simulink model "sst_cllc_ttype_inv_discrete"  (R2026b)
settings: Solver=ode23tb  StopTime=simlength  FixedStep=tc  MaxStep=glb_time.tc
values from neighbouring files (symbols this model uses):
  param = sst_cllc_ttype_setup(param)    [init_model.m]
undefined symbols (not defined in the file or in its folder): afe_ctrl, glb_time, grid_emu, hwdata, omega_set, single_phase_inverter_ctrl, sst_num_of_modules
libraries: fl_lib x28, nesl_utility x16, discrete_time_low_pass_filter x4, lithium_ion_battery x2, cllc_dcx x2, dclink_for_three_levels x2, full_bridge_three_level_ttype_ideal_switch_based_model x2, full_bridge_three_level_ttype_mosfet_based_model x2, simulink x2, cstblocks_lti x2, single_phase_three_levels_PWM_modulator x2, dq_vector_pi x2
(part 2 of 3)

== system sst_cllc_ttype_inv_discrete/single_phase_inverter_modB/single phase afe ==
  gate_commands : Inport
  ideal_switch_based_three_level_inverter_ttype : full_bridge_three_level_ttype_ideal_switch_based_model/ideal_switch_based_three_level_inverter_ttype  Vth=ideal_switch.Vth  Ron=ideal_switch.Rds_on  Vdon_diode=ideal_switch.Vdon_diode  Rdon_diode=ideal_switch.Rdon_diode  Csnubber=ideal_switch.Csnubber  Rsnubber=ideal_switch.Rsnubber
  mosfet_based_three_level_inverter_ttype : full_bridge_three_level_ttype_mosfet_based_model/mosfet_based_three_level_inverter_ttype  Commented=on  Vth_m=mosfet.inv.Vth  Rds_on_m=mosfet.inv.Rds_on  Eon_m=mosfet.inv.Eon  Eoff_m=mosfet.inv.Eoff  Erec_m=mosfet.inv.Err  Ion_sw_loss_m=mosfet.inv.Ion_sw_losses  Voff_sw_loss_m=mosfet.inv.Voff_sw_losses  Vdon_diode_m=mosfet.inv.Vdon_diode  Rdon_diode_m=mosfet.inv.Rdon_diode  rth_mosfet_JH_m=mosfet.inv.Rth_mosfet_JH  rth_mosfet_HA_m=heatsink.Rth_mosfet_HA  Csnubber_m=mosfet.inv.Csnubber  Rsnubber_m=mosfet.inv.Rsnubber  JunctionTermalMass_m=mosfet.inv.JunctionTermalMass  mass_heatsink_m=heatsink.no_weight  specific_heat_m=heatsink.cp  Tambient_m=heatsink.Tambient  DThs_init_m=heatsink.DThs_init  tc_m=glb_time.tc
  references : Subsystem  Commented=on
  uac_out(+) : PMIOPort  Side=Left
  uac_out(-) : PMIOPort  Port=2  Side=Left
  udc(+) : PMIOPort  Port=3  Side=Right
  np : PMIOPort  Port=4  Side=Right
  udc(-) : PMIOPort  Port=5  Side=Right
  wires:
  mosfet_based_three_level_inverter_ttype/1 -> references/1(m)
  gate_commands/1 -> ideal_switch_based_three_level_inverter_ttype/1, mosfet_based_three_level_inverter_ttype/1
  connections:
  np/RConn1 -- mosfet_based_three_level_inverter_ttype/RConn2 -- ideal_switch_based_three_level_inverter_ttype/RConn2
  udc(-)/RConn1 -- mosfet_based_three_level_inverter_ttype/RConn3 -- ideal_switch_based_three_level_inverter_ttype/RConn3
  uac_out(+)/RConn1 -- mosfet_based_three_level_inverter_ttype/LConn1 -- ideal_switch_based_three_level_inverter_ttype/LConn1
  udc(+)/RConn1 -- mosfet_based_three_level_inverter_ttype/RConn1 -- ideal_switch_based_three_level_inverter_ttype/RConn1
  uac_out(-)/RConn1 -- mosfet_based_three_level_inverter_ttype/LConn2 -- ideal_switch_based_three_level_inverter_ttype/LConn2

== system sst_cllc_ttype_inv_discrete/single_phase_inverter_modB/single phase inverter control ==
  acquisition_and_scaling_current_with_white_noise : Subsystem
  acquisition_and_scaling_dc_voltage : Subsystem
  acquisition_and_scaling_grid_voltage_ac : Subsystem
  acquisition_and_scaling_voltage : Subsystem
  inverter_current_output_pu_reference : Subsystem
  pwm modulator : Subsystem
  single_phase_inverter_ctrl : Subsystem
  gate_cmds : Outport
  tag scope: afe_phase_grid_hat_modB=global
  wires:
  single_phase_inverter_ctrl/2(phase_grid_hat) -> [afe_phase_grid_hat_modB]
  acquisition_and_scaling_grid_voltage_ac/1(out) -> single_phase_inverter_ctrl/6(ugrid_pu)  "ug_abc"
  [ac_grid_voltage] -> acquisition_and_scaling_grid_voltage_ac/1(in)
  [time_afe_module_B] -> single_phase_inverter_ctrl/5(local_time)
  acquisition_and_scaling_dc_voltage/1(out) -> single_phase_inverter_ctrl/4(dclink_voltage_pu)  "dclink_voltage_pu"
  [dclink_voltage_modB] -> acquisition_and_scaling_dc_voltage/1(in)
  inverter_current_output_pu_reference/1(afe_current_output_pu_reference) -> single_phase_inverter_ctrl/3(afe_current output_pu_reference)  "afe_current_output_pu_reference"
  acquisition_and_scaling_voltage/1(out) -> single_phase_inverter_ctrl/1(afe_voltage_output_pu)  "afe_voltage_output_pu"
  acquisition_and_scaling_current_with_white_noise/1(out) -> single_phase_inverter_ctrl/2(afe_current_output_pu)  "afe_current_output_pu"
  single_phase_inverter_ctrl/1(u_ctrl_out) -> pwm modulator/1(vout)
  [afe_voltage_output_modB] -> acquisition_and_scaling_voltage/1(in)
  [TRGO_AFE_modB] -> single_phase_inverter_ctrl/Trigger
  pwm modulator/1(gate_cmds) -> gate_cmds/1
  [afe_is_modB] -> acquisition_and_scaling_current_with_white_noise/1(in)
  [udq_ctrl_out_modA] -> single_phase_inverter_ctrl/7(udq_ctrl_out)

== system sst_cllc_ttype_inv_discrete/single_phase_inverter_modA/dclink/references ==
  m : Inport
  Bus Selector : BusSelector  OutputSignals=udc,udc_p_gnd,udc_n_gnd,Cdc1_current
  Bus Selector1 : BusSelector  OutputSignals=idc1,idc2
  tag scope: CFi_dc_current_modA=global, dclink_n2gnd_voltage_modA=global, dclink_p2gnd_voltage_modA=global, dclink_voltage_modA=global, idc1_m_modA=global, idc2_m_modA=global
  wires:
  m/1 -> Bus Selector/1, Bus Selector1/1
  Bus Selector1/1 -> [idc1_m_modA]  "<idc1>"
  Bus Selector/1 -> [dclink_voltage_modA]  "<udc>"
  Bus Selector/4 -> [CFi_dc_current_modA]  "<Cdc1_current>"
  Bus Selector/3 -> [dclink_n2gnd_voltage_modA]  "<udc_n_gnd>"
  Bus Selector/2 -> [dclink_p2gnd_voltage_modA]  "<udc_p_gnd>"
  Bus Selector1/2 -> [idc2_m_modA]  "<idc2>"

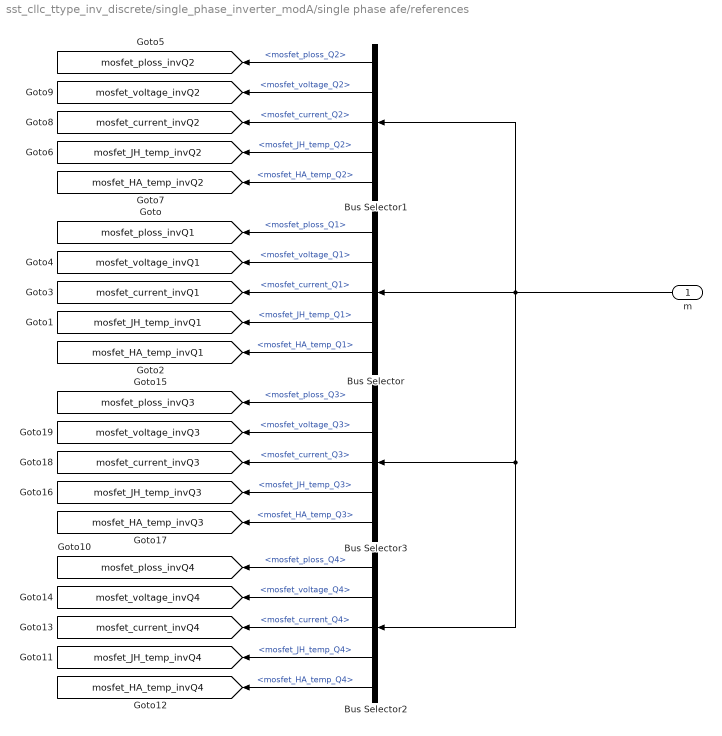
== system sst_cllc_ttype_inv_discrete/single_phase_inverter_modA/single phase afe/references ==
  m : Inport
  Bus Selector : BusSelector  OutputSignals=phaseleg_u.mosfet_ploss_Q1,phaseleg_u.mosfet_voltage_Q1,phaseleg_u.mosfet_current_Q1,phaseleg_u.mosfet_JH_temp_Q1,phaseleg_u.mosfet_HA_temp_Q1
  Bus Selector1 : BusSelector  OutputSignals=phaseleg_u.mosfet_ploss_Q2,phaseleg_u.mosfet_voltage_Q2,phaseleg_u.mosfet_current_Q2,phaseleg_u.mosfet_JH_temp_Q2,phaseleg_u.mosfet_HA_temp_Q2
  Bus Selector2 : BusSelector  OutputSignals=phaseleg_u.mosfet_ploss_Q4,phaseleg_u.mosfet_voltage_Q4,phaseleg_u.mosfet_current_Q4,phaseleg_u.mosfet_JH_temp_Q4,phaseleg_u.mosfet_HA_temp_Q4
  Bus Selector3 : BusSelector  OutputSignals=phaseleg_u.mosfet_ploss_Q3,phaseleg_u.mosfet_voltage_Q3,phaseleg_u.mosfet_current_Q3,phaseleg_u.mosfet_JH_temp_Q3,phaseleg_u.mosfet_HA_temp_Q3
  tag scope: mosfet_HA_temp_invQ1=global, mosfet_HA_temp_invQ2=global, mosfet_HA_temp_invQ3=global, mosfet_HA_temp_invQ4=global, mosfet_JH_temp_invQ1=global, mosfet_JH_temp_invQ2=global, mosfet_JH_temp_invQ3=global, mosfet_JH_temp_invQ4=global, mosfet_current_invQ1=global, mosfet_current_invQ2=global, mosfet_current_invQ3=global, mosfet_current_invQ4=global, mosfet_ploss_invQ1=global, mosfet_ploss_invQ2=global, mosfet_ploss_invQ3=global, mosfet_ploss_invQ4=global, mosfet_voltage_invQ1=global, mosfet_voltage_invQ2=global, mosfet_voltage_invQ3=global, mosfet_voltage_invQ4=global
  wires:
  Bus Selector/4 -> [mosfet_JH_temp_invQ1]  "<mosfet_JH_temp_Q1>"
  Bus Selector3/5 -> [mosfet_HA_temp_invQ3]  "<mosfet_HA_temp_Q3>"
  Bus Selector1/1 -> [mosfet_ploss_invQ2]  "<mosfet_ploss_Q2>"
  Bus Selector/5 -> [mosfet_HA_temp_invQ1]  "<mosfet_HA_temp_Q1>"
  Bus Selector/2 -> [mosfet_voltage_invQ1]  "<mosfet_voltage_Q1>"
  Bus Selector2/2 -> [mosfet_voltage_invQ4]  "<mosfet_voltage_Q4>"
  Bus Selector3/3 -> [mosfet_current_invQ3]  "<mosfet_current_Q3>"
  Bus Selector3/2 -> [mosfet_voltage_invQ3]  "<mosfet_voltage_Q3>"
  Bus Selector3/1 -> [mosfet_ploss_invQ3]  "<mosfet_ploss_Q3>"
  Bus Selector2/1 -> [mosfet_ploss_invQ4]  "<mosfet_ploss_Q4>"
  Bus Selector2/5 -> [mosfet_HA_temp_invQ4]  "<mosfet_HA_temp_Q4>"
  m/1 -> Bus Selector2/1, Bus Selector3/1, Bus Selector/1, Bus Selector1/1
  Bus Selector1/2 -> [mosfet_voltage_invQ2]  "<mosfet_voltage_Q2>"
  Bus Selector2/3 -> [mosfet_current_invQ4]  "<mosfet_current_Q4>"
  Bus Selector2/4 -> [mosfet_JH_temp_invQ4]  "<mosfet_JH_temp_Q4>"
  Bus Selector1/4 -> [mosfet_JH_temp_invQ2]  "<mosfet_JH_temp_Q2>"
  Bus Selector/1 -> [mosfet_ploss_invQ1]  "<mosfet_ploss_Q1>"
  Bus Selector1/3 -> [mosfet_current_invQ2]  "<mosfet_current_Q2>"
  Bus Selector3/4 -> [mosfet_JH_temp_invQ3]  "<mosfet_JH_temp_Q3>"
  Bus Selector/3 -> [mosfet_current_invQ1]  "<mosfet_current_Q1>"
  Bus Selector1/5 -> [mosfet_HA_temp_invQ2]  "<mosfet_HA_temp_Q2>"

== system sst_cllc_ttype_inv_discrete/single_phase_inverter_modA/single phase inverter control/acquisition_and_scaling_current ==
  in : Inport
  1/Ti5 : Gain  Gain=1/hwdata.single_phase_inverter.ibez  SaturateOnIntegerOverflow=on  OutDataTypeStr=Inherit: Same as input  ParamDataTypeStr=Inherit: Same as input
  Quantizer : Quantizer  QuantizationInterval=adc11_quantization
  out : Outport
  wires:
  Quantizer/1 -> out/1
  1/Ti5/1 -> Quantizer/1
  in/1 -> 1/Ti5/1

== system sst_cllc_ttype_inv_discrete/single_phase_inverter_modA/single phase inverter control/acquisition_and_scaling_current_with_white_noise ==
  in : Inport
  1/Ti5 : Gain  Gain=1/hwdata.single_phase_inverter.ibez  SaturateOnIntegerOverflow=on  OutDataTypeStr=Inherit: Same as input  ParamDataTypeStr=Inherit: Same as input
  Band-Limited White Noise : simulink/Sources/Band-Limited White Noise  Commented=on  Cov=1e-10  Ts=glb_time.tc  seed=[23341]
  Quantizer : Quantizer  QuantizationInterval=adc12_quantization
  Sum : Sum  Inputs=|++
  current_measure_with-without noise : Scope  NumInputPorts=2
      settings: ActiveDisplayYMinimum=-42.907449410116151  ActiveDisplayYMaximum=14.197534402303543  DataLoggingVariableName=ScopeData15
  out : Outport
  wires:
  1/Ti5/1 -> current_measure_with-without noise/1, Sum/1  "iload_without_noise"
  Sum/1 -> Quantizer/1
  Band-Limited White Noise/1 -> Sum/2
  Quantizer/1 -> out/1, current_measure_with-without noise/2  "iload_with_noise"
  in/1 -> 1/Ti5/1

== system sst_cllc_ttype_inv_discrete/single_phase_inverter_modA/single phase inverter control/acquisition_and_scaling_dc_voltage ==
  in : Inport
  1/Ti3 : Gain  Gain=1/hwdata.single_phase_inverter.udc_nom  SaturateOnIntegerOverflow=on  OutDataTypeStr=Inherit: Same as input  ParamDataTypeStr=Inherit: Same as input
  Quantizer : Quantizer  QuantizationInterval=adc12_quantization
  out : Outport
  wires:
  in/1 -> 1/Ti3/1
  1/Ti3/1 -> Quantizer/1
  Quantizer/1 -> out/1

== system sst_cllc_ttype_inv_discrete/single_phase_inverter_modA/single phase inverter control/acquisition_and_scaling_grid_voltage_ac ==
  in : Inport
  1/Ti1 : Gain  Gain=sst_num_of_modules  SaturateOnIntegerOverflow=on  OutDataTypeStr=Inherit: Same as input  ParamDataTypeStr=Inherit: Same as input
  1/Ti5 : Gain  Gain=1/grid_emu.u2bez  SaturateOnIntegerOverflow=on  OutDataTypeStr=Inherit: Same as input  ParamDataTypeStr=Inherit: Same as input
  Quantizer : Quantizer  QuantizationInterval=adc12_quantization
  out : Outport
  wires:
  Quantizer/1 -> out/1
  1/Ti5/1 -> Quantizer/1
  in/1 -> 1/Ti1/1
  1/Ti1/1 -> 1/Ti5/1

== system sst_cllc_ttype_inv_discrete/single_phase_inverter_modA/single phase inverter control/acquisition_and_scaling_voltage ==
  in : Inport
  1/Ti5 : Gain  Gain=1/hwdata.single_phase_inverter.ubez  SaturateOnIntegerOverflow=on  OutDataTypeStr=Inherit: Same as input  ParamDataTypeStr=Inherit: Same as input
  Quantizer : Quantizer  QuantizationInterval=adc12_quantization
  pwm filtering for measure : cstblocks_lti/LTI System  sys=sogi.flt.beta  IC=[]  PadeOrder=0
  out : Outport
  wires:
  in/1 -> 1/Ti5/1
  pwm filtering for measure/1 -> Quantizer/1
  1/Ti5/1 -> pwm filtering for measure/1
  Quantizer/1 -> out/1

== system sst_cllc_ttype_inv_discrete/single_phase_inverter_modA/single phase inverter control/inverter_current_output_pu_reference ==
  Rate Limiter : RateLimiter  RisingSlewLimit=param.spinv.i_ref_slew  FallingSlewLimit=-param.spinv.i_ref_slew  SampleTimeMode=inherited
  Step : Step  Time=param.spinv.t_ref  FinalValue=param.spinv.i_ref  SampleTime=0
  afe_current_output_pu_reference : Outport
  wires:
  Step/1 -> Rate Limiter/1
  Rate Limiter/1 -> afe_current_output_pu_reference/1

== system sst_cllc_ttype_inv_discrete/single_phase_inverter_modA/single phase inverter control/pwm modulator ==
  vout : Inport
  Constant : Constant  Value=0
  single_phase_three_levels_PWM_generator_with_global_TRGO : single_phase_three_levels_PWM_modulator/single_phase_three_levels_PWM_generator_with_global_TRGO  f=glb_time.fPWM_INV  m_up=1  m_low=-1  dead_time=glb_time.dead_time_AFE  pos_cmd_gate=15  neg_cmd_gate=-10  polarity=1  tc=glb_time.tc  double_sampling=glb_time.TRGO_AFE_double_update
  gate_cmds : Outport
  tag scope: TRGO_AFE_modA=global
  wires:
  vout/1 -> single_phase_three_levels_PWM_generator_with_global_TRGO/3
  Constant/1 -> single_phase_three_levels_PWM_generator_with_global_TRGO/2
  single_phase_three_levels_PWM_generator_with_global_TRGO/2 -> gate_cmds/1
  single_phase_three_levels_PWM_generator_with_global_TRGO/1 -> [TRGO_AFE_modA]
  [time_afe_module_A] -> single_phase_three_levels_PWM_generator_with_global_TRGO/1

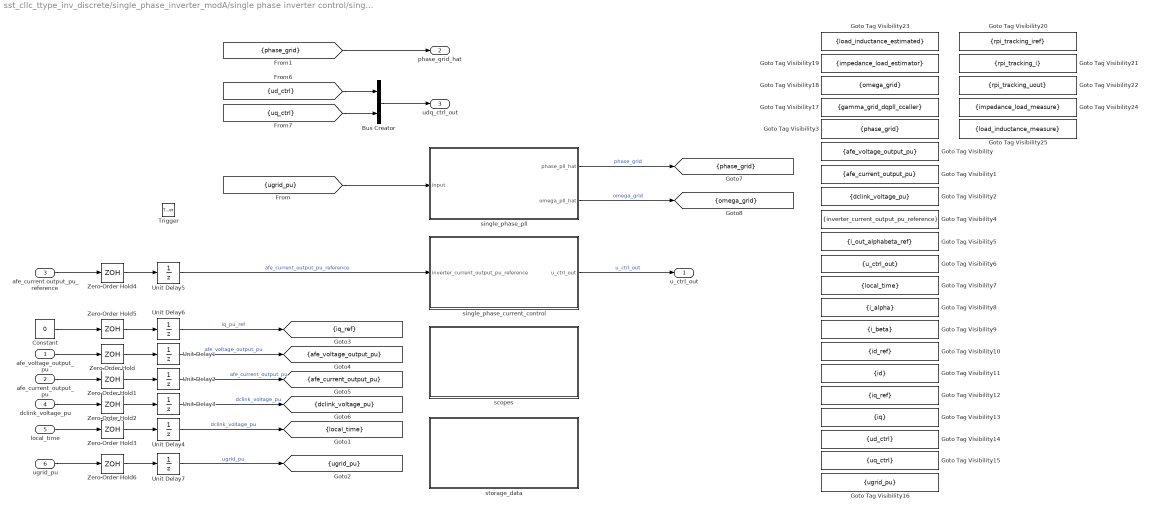
== system sst_cllc_ttype_inv_discrete/single_phase_inverter_modA/single phase inverter control/single_phase_inverter_ctrl ==
  afe_voltage_output_pu : Inport
  afe_current_output_pu : Inport  Port=2
  afe_current output_pu_reference : Inport  Port=3
  dclink_voltage_pu : Inport  Port=4
  local_time : Inport  Port=5
  ugrid_pu : Inport  Port=6
  Trigger : TriggerPort  VariantControl=(inherit)  PortDimensions=1
  Bus Creator : BusCreator  Inputs=2
  Constant : Constant  Value=0
  Goto Tag Visibility : GotoTagVisibility  GotoTag=afe_voltage_output_pu
  Goto Tag Visibility1 : GotoTagVisibility  GotoTag=afe_current_output_pu
  Goto Tag Visibility10 : GotoTagVisibility  GotoTag=id_ref
  Goto Tag Visibility11 : GotoTagVisibility  GotoTag=id
  Goto Tag Visibility12 : GotoTagVisibility  GotoTag=iq_ref
  Goto Tag Visibility13 : GotoTagVisibility  GotoTag=iq
  Goto Tag Visibility14 : GotoTagVisibility  GotoTag=ud_ctrl
  Goto Tag Visibility15 : GotoTagVisibility  GotoTag=uq_ctrl
  Goto Tag Visibility16 : GotoTagVisibility  GotoTag=ugrid_pu
  Goto Tag Visibility17 : GotoTagVisibility  GotoTag=gamma_grid_dqpll_ccaller
  Goto Tag Visibility18 : GotoTagVisibility  GotoTag=omega_grid
  Goto Tag Visibility19 : GotoTagVisibility  GotoTag=impedance_load_estimator
  Goto Tag Visibility2 : GotoTagVisibility  GotoTag=dclink_voltage_pu
  Goto Tag Visibility20 : GotoTagVisibility  GotoTag=rpi_tracking_iref
  Goto Tag Visibility21 : GotoTagVisibility  GotoTag=rpi_tracking_i
  Goto Tag Visibility22 : GotoTagVisibility  GotoTag=rpi_tracking_uout
  Goto Tag Visibility23 : GotoTagVisibility  GotoTag=load_inductance_estimated
  Goto Tag Visibility24 : GotoTagVisibility  GotoTag=impedance_load_measure
  Goto Tag Visibility25 : GotoTagVisibility  GotoTag=load_inductance_measure
  Goto Tag Visibility3 : GotoTagVisibility  GotoTag=phase_grid
  Goto Tag Visibility4 : GotoTagVisibility  GotoTag=inverter_current_output_pu_reference
  Goto Tag Visibility5 : GotoTagVisibility  GotoTag=i_out_alphabeta_ref
  Goto Tag Visibility6 : GotoTagVisibility  GotoTag=u_ctrl_out
  Goto Tag Visibility7 : GotoTagVisibility  GotoTag=local_time
  Goto Tag Visibility8 : GotoTagVisibility  GotoTag=i_alpha
  Goto Tag Visibility9 : GotoTagVisibility  GotoTag=i_beta
  Unit Delay{1..7} (7 alike) : UnitDelay  SampleTime=-1
  Zero-Order Hold{,1..6} (7 alike) : ZeroOrderHold  SampleTime=-1
  scopes : Subsystem
  single_phase_current_control : Subsystem
  single_phase_pll : Subsystem
  storage_data : Subsystem
  u_ctrl_out : Outport
  phase_grid_hat : Outport  Port=2
  udq_ctrl_out : Outport  Port=3
  tag scope: afe_current_output_pu=scoped, afe_voltage_output_pu=scoped, dclink_voltage_pu=scoped, iq_ref=scoped, local_time=scoped, omega_grid=scoped, phase_grid=scoped, ugrid_pu=scoped
  wires:
  afe_voltage_output_pu/1 -> Zero-Order Hold/1
  afe_current_output_pu/1 -> Zero-Order Hold1/1
  dclink_voltage_pu/1 -> Zero-Order Hold2/1
  Unit Delay1/1 -> [afe_voltage_output_pu]  "afe_voltage_output_pu"
  Unit Delay2/1 -> [afe_current_output_pu]  "afe_current_output_pu"
  Unit Delay3/1 -> [dclink_voltage_pu]  "dclink_voltage_pu"
  single_phase_pll/1(phase_pll_hat) -> [phase_grid]  "phase_grid"
  afe_current output_pu_reference/1 -> Zero-Order Hold4/1
  single_phase_current_control/1(u_ctrl_out) -> u_ctrl_out/1  "u_ctrl_out"
  Zero-Order Hold/1 -> Unit Delay1/1
  Zero-Order Hold1/1 -> Unit Delay2/1
  Zero-Order Hold2/1 -> Unit Delay3/1
  Zero-Order Hold3/1 -> Unit Delay4/1
  Unit Delay4/1 -> [local_time]  "dclink_voltage_pu"
  local_time/1 -> Zero-Order Hold3/1
  Zero-Order Hold4/1 -> Unit Delay5/1
  Unit Delay5/1 -> single_phase_current_control/1(inverter_current_output_pu_reference)  "afe_current_output_pu_reference"
  Constant/1 -> Zero-Order Hold5/1
  Zero-Order Hold5/1 -> Unit Delay6/1
  Unit Delay6/1 -> [iq_ref]  "iq_pu_ref"
  ugrid_pu/1 -> Zero-Order Hold6/1
  Zero-Order Hold6/1 -> Unit Delay7/1
  Unit Delay7/1 -> [ugrid_pu]  "ugrid_pu"
  single_phase_pll/2(omega_pll_hat) -> [omega_grid]  "omega_grid"
  [ugrid_pu] -> single_phase_pll/1(input)
  [phase_grid] -> phase_grid_hat/1
  Bus Creator/1 -> udq_ctrl_out/1
  [ud_ctrl] -> Bus Creator/1
  [uq_ctrl] -> Bus Creator/2

== system sst_cllc_ttype_inv_discrete/single_phase_inverter_modB/dclink/references ==
  m : Inport
  Bus Selector : BusSelector  OutputSignals=udc,udc_p_gnd,udc_n_gnd,Cdc1_current
  Bus Selector1 : BusSelector  OutputSignals=idc1,idc2
  tag scope: CFi_dc_current_modB=global, dclink_n2gnd_voltage_modB=global, dclink_p2gnd_voltage_modB=global, dclink_voltage_modB=global, idc1_m_modB=global, idc2_m_modB=global
  wires:
  Bus Selector1/2 -> [idc2_m_modB]  "<idc2>"
  Bus Selector/2 -> [dclink_p2gnd_voltage_modB]  "<udc_p_gnd>"
  Bus Selector/3 -> [dclink_n2gnd_voltage_modB]  "<udc_n_gnd>"
  Bus Selector/4 -> [CFi_dc_current_modB]  "<Cdc1_current>"
  Bus Selector/1 -> [dclink_voltage_modB]  "<udc>"
  Bus Selector1/1 -> [idc1_m_modB]  "<idc1>"
  m/1 -> Bus Selector1/1, Bus Selector/1

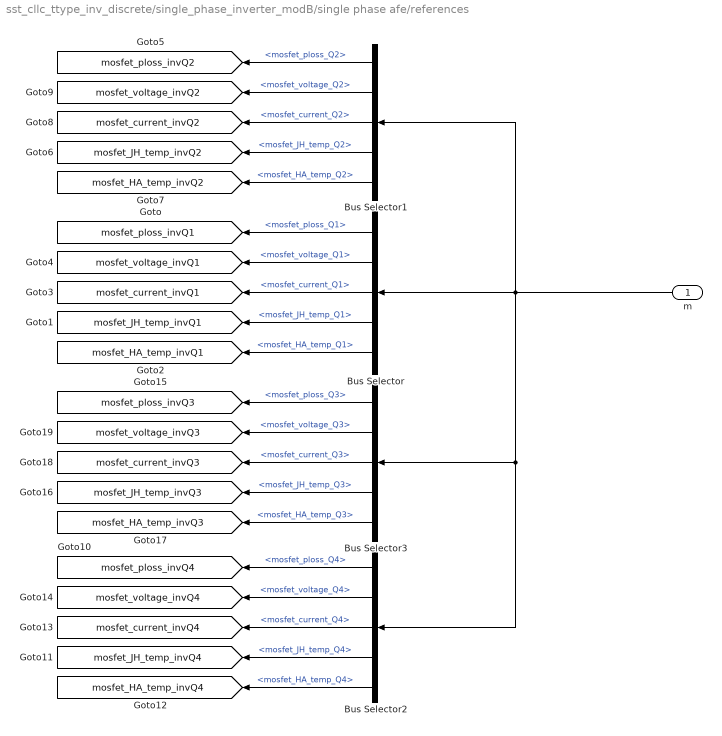
== system sst_cllc_ttype_inv_discrete/single_phase_inverter_modB/single phase afe/references ==
  m : Inport
  Bus Selector : BusSelector  OutputSignals=phaseleg_u.mosfet_ploss_Q1,phaseleg_u.mosfet_voltage_Q1,phaseleg_u.mosfet_current_Q1,phaseleg_u.mosfet_JH_temp_Q1,phaseleg_u.mosfet_HA_temp_Q1
  Bus Selector1 : BusSelector  OutputSignals=phaseleg_u.mosfet_ploss_Q2,phaseleg_u.mosfet_voltage_Q2,phaseleg_u.mosfet_current_Q2,phaseleg_u.mosfet_JH_temp_Q2,phaseleg_u.mosfet_HA_temp_Q2
  Bus Selector2 : BusSelector  OutputSignals=phaseleg_u.mosfet_ploss_Q4,phaseleg_u.mosfet_voltage_Q4,phaseleg_u.mosfet_current_Q4,phaseleg_u.mosfet_JH_temp_Q4,phaseleg_u.mosfet_HA_temp_Q4
  Bus Selector3 : BusSelector  OutputSignals=phaseleg_u.mosfet_ploss_Q3,phaseleg_u.mosfet_voltage_Q3,phaseleg_u.mosfet_current_Q3,phaseleg_u.mosfet_JH_temp_Q3,phaseleg_u.mosfet_HA_temp_Q3
  tag scope: mosfet_HA_temp_invQ1=global, mosfet_HA_temp_invQ2=global, mosfet_HA_temp_invQ3=global, mosfet_HA_temp_invQ4=global, mosfet_JH_temp_invQ1=global, mosfet_JH_temp_invQ2=global, mosfet_JH_temp_invQ3=global, mosfet_JH_temp_invQ4=global, mosfet_current_invQ1=global, mosfet_current_invQ2=global, mosfet_current_invQ3=global, mosfet_current_invQ4=global, mosfet_ploss_invQ1=global, mosfet_ploss_invQ2=global, mosfet_ploss_invQ3=global, mosfet_ploss_invQ4=global, mosfet_voltage_invQ1=global, mosfet_voltage_invQ2=global, mosfet_voltage_invQ3=global, mosfet_voltage_invQ4=global
  wires:
  Bus Selector1/5 -> [mosfet_HA_temp_invQ2]  "<mosfet_HA_temp_Q2>"
  Bus Selector/3 -> [mosfet_current_invQ1]  "<mosfet_current_Q1>"
  Bus Selector3/4 -> [mosfet_JH_temp_invQ3]  "<mosfet_JH_temp_Q3>"
  Bus Selector1/3 -> [mosfet_current_invQ2]  "<mosfet_current_Q2>"
  Bus Selector/1 -> [mosfet_ploss_invQ1]  "<mosfet_ploss_Q1>"
  Bus Selector1/4 -> [mosfet_JH_temp_invQ2]  "<mosfet_JH_temp_Q2>"
  Bus Selector2/4 -> [mosfet_JH_temp_invQ4]  "<mosfet_JH_temp_Q4>"
  Bus Selector2/3 -> [mosfet_current_invQ4]  "<mosfet_current_Q4>"
  Bus Selector1/2 -> [mosfet_voltage_invQ2]  "<mosfet_voltage_Q2>"
  m/1 -> Bus Selector1/1, Bus Selector/1, Bus Selector3/1, Bus Selector2/1
  Bus Selector2/5 -> [mosfet_HA_temp_invQ4]  "<mosfet_HA_temp_Q4>"
  Bus Selector2/1 -> [mosfet_ploss_invQ4]  "<mosfet_ploss_Q4>"
  Bus Selector3/1 -> [mosfet_ploss_invQ3]  "<mosfet_ploss_Q3>"
  Bus Selector3/2 -> [mosfet_voltage_invQ3]  "<mosfet_voltage_Q3>"
  Bus Selector3/3 -> [mosfet_current_invQ3]  "<mosfet_current_Q3>"
  Bus Selector2/2 -> [mosfet_voltage_invQ4]  "<mosfet_voltage_Q4>"
  Bus Selector/2 -> [mosfet_voltage_invQ1]  "<mosfet_voltage_Q1>"
  Bus Selector/5 -> [mosfet_HA_temp_invQ1]  "<mosfet_HA_temp_Q1>"
  Bus Selector1/1 -> [mosfet_ploss_invQ2]  "<mosfet_ploss_Q2>"
  Bus Selector3/5 -> [mosfet_HA_temp_invQ3]  "<mosfet_HA_temp_Q3>"
  Bus Selector/4 -> [mosfet_JH_temp_invQ1]  "<mosfet_JH_temp_Q1>"

== system sst_cllc_ttype_inv_discrete/single_phase_inverter_modB/single phase inverter control/acquisition_and_scaling_current_with_white_noise ==
  in : Inport
  1/Ti5 : Gain  Gain=1/hwdata.single_phase_inverter.ibez  SaturateOnIntegerOverflow=on  OutDataTypeStr=Inherit: Same as input  ParamDataTypeStr=Inherit: Same as input
  Band-Limited White Noise : simulink/Sources/Band-Limited White Noise  Commented=on  Cov=1e-10  Ts=glb_time.tc  seed=[23341]
  Quantizer : Quantizer  QuantizationInterval=adc12_quantization
  Sum : Sum  Inputs=|++
  current_measure_with-without noise : Scope  NumInputPorts=2
      settings: ActiveDisplayYMinimum=-42.907449410116151  ActiveDisplayYMaximum=14.197534402303543  DataLoggingVariableName=ScopeData15
  out : Outport
  wires:
  in/1 -> 1/Ti5/1
  Quantizer/1 -> current_measure_with-without noise/2, out/1  "iload_with_noise"
  Band-Limited White Noise/1 -> Sum/2
  Sum/1 -> Quantizer/1
  1/Ti5/1 -> Sum/1, current_measure_with-without noise/1  "iload_without_noise"

== system sst_cllc_ttype_inv_discrete/single_phase_inverter_modB/single phase inverter control/acquisition_and_scaling_dc_voltage ==
  in : Inport
  1/Ti3 : Gain  Gain=1/hwdata.single_phase_inverter.udc_nom  SaturateOnIntegerOverflow=on  OutDataTypeStr=Inherit: Same as input  ParamDataTypeStr=Inherit: Same as input
  Quantizer : Quantizer  QuantizationInterval=adc12_quantization
  out : Outport
  wires:
  Quantizer/1 -> out/1
  1/Ti3/1 -> Quantizer/1
  in/1 -> 1/Ti3/1

== system sst_cllc_ttype_inv_discrete/single_phase_inverter_modB/single phase inverter control/acquisition_and_scaling_grid_voltage_ac ==
  in : Inport
  1/Ti1 : Gain  Gain=sst_num_of_modules  SaturateOnIntegerOverflow=on  OutDataTypeStr=Inherit: Same as input  ParamDataTypeStr=Inherit: Same as input
  1/Ti5 : Gain  Gain=1/grid_emu.u2bez  SaturateOnIntegerOverflow=on  OutDataTypeStr=Inherit: Same as input  ParamDataTypeStr=Inherit: Same as input
  Quantizer : Quantizer  QuantizationInterval=adc12_quantization
  out : Outport
  wires:
  in/1 -> 1/Ti1/1
  1/Ti5/1 -> Quantizer/1
  Quantizer/1 -> out/1
  1/Ti1/1 -> 1/Ti5/1

== system sst_cllc_ttype_inv_discrete/single_phase_inverter_modB/single phase inverter control/acquisition_and_scaling_voltage ==
  in : Inport
  1/Ti5 : Gain  Gain=1/hwdata.single_phase_inverter.ubez  SaturateOnIntegerOverflow=on  OutDataTypeStr=Inherit: Same as input  ParamDataTypeStr=Inherit: Same as input
  Quantizer : Quantizer  QuantizationInterval=adc12_quantization
  pwm filtering for measure : cstblocks_lti/LTI System  sys=sogi.flt.beta  IC=[]  PadeOrder=0
  out : Outport
  wires:
  Quantizer/1 -> out/1
  1/Ti5/1 -> pwm filtering for measure/1
  pwm filtering for measure/1 -> Quantizer/1
  in/1 -> 1/Ti5/1

== system sst_cllc_ttype_inv_discrete/single_phase_inverter_modB/single phase inverter control/inverter_current_output_pu_reference ==
  Constant : Constant  Value=param.spinv.i_ref
  afe_current_output_pu_reference : Outport
  wires:
  Constant/1 -> afe_current_output_pu_reference/1

== system sst_cllc_ttype_inv_discrete/single_phase_inverter_modB/single phase inverter control/pwm modulator ==
  vout : Inport
  Constant : Constant  Value=0
  single_phase_three_levels_PWM_generator_with_global_TRGO : single_phase_three_levels_PWM_modulator/single_phase_three_levels_PWM_generator_with_global_TRGO  f=glb_time.fPWM_INV  m_up=1  m_low=-1  dead_time=glb_time.dead_time_AFE  pos_cmd_gate=15  neg_cmd_gate=-10  polarity=1  tc=glb_time.tc  double_sampling=glb_time.TRGO_AFE_double_update
  gate_cmds : Outport
  tag scope: TRGO_AFE_modB=global
  wires:
  [time_afe_module_B] -> single_phase_three_levels_PWM_generator_with_global_TRGO/1
  single_phase_three_levels_PWM_generator_with_global_TRGO/1 -> [TRGO_AFE_modB]
  single_phase_three_levels_PWM_generator_with_global_TRGO/2 -> gate_cmds/1
  Constant/1 -> single_phase_three_levels_PWM_generator_with_global_TRGO/2
  vout/1 -> single_phase_three_levels_PWM_generator_with_global_TRGO/3

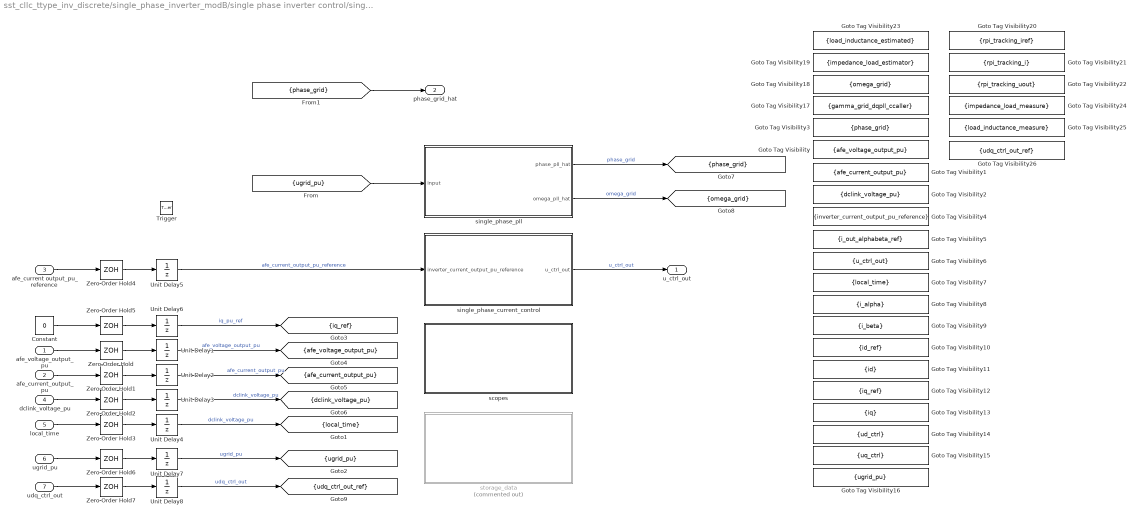
== system sst_cllc_ttype_inv_discrete/single_phase_inverter_modB/single phase inverter control/single_phase_inverter_ctrl ==
  afe_voltage_output_pu : Inport
  afe_current_output_pu : Inport  Port=2
  afe_current output_pu_reference : Inport  Port=3
  dclink_voltage_pu : Inport  Port=4
  local_time : Inport  Port=5
  ugrid_pu : Inport  Port=6
  udq_ctrl_out : Inport  Port=7
  Trigger : TriggerPort  VariantControl=(inherit)  PortDimensions=1
  Constant : Constant  Value=0
  Goto Tag Visibility : GotoTagVisibility  GotoTag=afe_voltage_output_pu
  Goto Tag Visibility1 : GotoTagVisibility  GotoTag=afe_current_output_pu
  Goto Tag Visibility10 : GotoTagVisibility  GotoTag=id_ref
  Goto Tag Visibility11 : GotoTagVisibility  GotoTag=id
  Goto Tag Visibility12 : GotoTagVisibility  GotoTag=iq_ref
  Goto Tag Visibility13 : GotoTagVisibility  GotoTag=iq
  Goto Tag Visibility14 : GotoTagVisibility  GotoTag=ud_ctrl
  Goto Tag Visibility15 : GotoTagVisibility  GotoTag=uq_ctrl
  Goto Tag Visibility16 : GotoTagVisibility  GotoTag=ugrid_pu
  Goto Tag Visibility17 : GotoTagVisibility  GotoTag=gamma_grid_dqpll_ccaller
  Goto Tag Visibility18 : GotoTagVisibility  GotoTag=omega_grid
  Goto Tag Visibility19 : GotoTagVisibility  GotoTag=impedance_load_estimator
  Goto Tag Visibility2 : GotoTagVisibility  GotoTag=dclink_voltage_pu
  Goto Tag Visibility20 : GotoTagVisibility  GotoTag=rpi_tracking_iref
  Goto Tag Visibility21 : GotoTagVisibility  GotoTag=rpi_tracking_i
  Goto Tag Visibility22 : GotoTagVisibility  GotoTag=rpi_tracking_uout
  Goto Tag Visibility23 : GotoTagVisibility  GotoTag=load_inductance_estimated
  Goto Tag Visibility24 : GotoTagVisibility  GotoTag=impedance_load_measure
  Goto Tag Visibility25 : GotoTagVisibility  GotoTag=load_inductance_measure
  Goto Tag Visibility26 : GotoTagVisibility  GotoTag=udq_ctrl_out_ref
  Goto Tag Visibility3 : GotoTagVisibility  GotoTag=phase_grid
  Goto Tag Visibility4 : GotoTagVisibility  GotoTag=inverter_current_output_pu_reference
  Goto Tag Visibility5 : GotoTagVisibility  GotoTag=i_out_alphabeta_ref
  Goto Tag Visibility6 : GotoTagVisibility  GotoTag=u_ctrl_out
  Goto Tag Visibility7 : GotoTagVisibility  GotoTag=local_time
  Goto Tag Visibility8 : GotoTagVisibility  GotoTag=i_alpha
  Goto Tag Visibility9 : GotoTagVisibility  GotoTag=i_beta
  Unit Delay{1..8} (8 alike) : UnitDelay  SampleTime=-1
  Zero-Order Hold{,1..7} (8 alike) : ZeroOrderHold  SampleTime=-1
  scopes : Subsystem
  single_phase_current_control : Subsystem
  single_phase_pll : Subsystem
  storage_data : Subsystem  Commented=on
  u_ctrl_out : Outport
  phase_grid_hat : Outport  Port=2
  tag scope: afe_current_output_pu=scoped, afe_voltage_output_pu=scoped, dclink_voltage_pu=scoped, iq_ref=scoped, local_time=scoped, omega_grid=scoped, phase_grid=scoped, udq_ctrl_out_ref=scoped, ugrid_pu=scoped
  wires:
  [phase_grid] -> phase_grid_hat/1
  [ugrid_pu] -> single_phase_pll/1(input)
  single_phase_pll/2(omega_pll_hat) -> [omega_grid]  "omega_grid"
  Unit Delay7/1 -> [ugrid_pu]  "ugrid_pu"
  Zero-Order Hold6/1 -> Unit Delay7/1
  ugrid_pu/1 -> Zero-Order Hold6/1
  Unit Delay6/1 -> [iq_ref]  "iq_pu_ref"
  Zero-Order Hold5/1 -> Unit Delay6/1
  Constant/1 -> Zero-Order Hold5/1
  Unit Delay5/1 -> single_phase_current_control/1(inverter_current_output_pu_reference)  "afe_current_output_pu_reference"
  Zero-Order Hold4/1 -> Unit Delay5/1
  local_time/1 -> Zero-Order Hold3/1
  Unit Delay4/1 -> [local_time]  "dclink_voltage_pu"
  Zero-Order Hold3/1 -> Unit Delay4/1
  Zero-Order Hold2/1 -> Unit Delay3/1
  Zero-Order Hold1/1 -> Unit Delay2/1
  Zero-Order Hold/1 -> Unit Delay1/1
  single_phase_current_control/1(u_ctrl_out) -> u_ctrl_out/1  "u_ctrl_out"
  afe_current output_pu_reference/1 -> Zero-Order Hold4/1
  single_phase_pll/1(phase_pll_hat) -> [phase_grid]  "phase_grid"
  Unit Delay3/1 -> [dclink_voltage_pu]  "dclink_voltage_pu"
  Unit Delay2/1 -> [afe_current_output_pu]  "afe_current_output_pu"
  Unit Delay1/1 -> [afe_voltage_output_pu]  "afe_voltage_output_pu"
  dclink_voltage_pu/1 -> Zero-Order Hold2/1
  afe_current_output_pu/1 -> Zero-Order Hold1/1
  afe_voltage_output_pu/1 -> Zero-Order Hold/1
  udq_ctrl_out/1 -> Zero-Order Hold7/1
  Zero-Order Hold7/1 -> Unit Delay8/1
  Unit Delay8/1 -> [udq_ctrl_out_ref]  "udq_ctrl_out"

== system sst_cllc_ttype_inv_discrete/single_phase_inverter_modA/single phase inverter control/single_phase_inverter_ctrl/scopes ==
  Bus Creator1 : BusCreator  Inputs=3
  Bus Creator2 : BusCreator  Inputs=2
  Bus Creator3 : BusCreator  Inputs=2
  Bus Creator4 : BusCreator  Inputs=2
  single phase inverter tracking current scope 1 : Scope  NumInputPorts=2
      settings: ActiveDisplayYMinimum=-0.98089599609375  ActiveDisplayYMaximum=0.98138427734375  DataLoggingVariableName=ScopeData12
  single phase inverter tracking current scope 2 : Scope  NumInputPorts=2
      settings: ActiveDisplayYMinimum=-1.2603759765625  ActiveDisplayYMaximum=1.2652587890625  DataLoggingVariableName=ScopeData2
  wires:
  Bus Creator1/1 -> single phase inverter tracking current scope 1/2  "is_tracking"
  [i_out_alphabeta_ref] -> Bus Creator1/2  "i_out_inverter_pu_ref"
  [afe_current_output_pu] -> Bus Creator1/3  "inverter_current_output_pu"
  [afe_voltage_output_pu] -> Bus Creator2/1  "inverter_voltage_output_pu"
  Bus Creator2/1 -> single phase inverter tracking current scope 1/1  "load"
  [inverter_current_output_pu_reference] -> Bus Creator1/1  "inverter_current_output_pu_reference"
  [afe_current_output_pu] -> Bus Creator2/2  "inverter_current_output_pu"
  [u_ctrl_out] -> Bus Creator3/1  "u_ctrl_out"
  [afe_voltage_output_pu] -> Bus Creator3/2  "inverter_voltage_output_pu"
  Bus Creator3/1 -> single phase inverter tracking current scope 2/2  "u_load"
  [afe_current_output_pu] -> Bus Creator4/2  "inverter_current_output_pu"
  [i_out_alphabeta_ref] -> Bus Creator4/1  "i_out_alphabeta_ref"
  Bus Creator4/1 -> single phase inverter tracking current scope 2/1  "i_load"

== system sst_cllc_ttype_inv_discrete/single_phase_inverter_modA/single phase inverter control/single_phase_inverter_ctrl/single_phase_current_control ==
  inverter_current_output_pu_reference : Inport
  current_reference_generation : Subsystem
  dqpi_current_controller : Subsystem
  u_ctrl_out : Outport
  tag scope: i_out_alphabeta_ref=scoped, inverter_current_output_pu_reference=scoped, u_ctrl_out=scoped
  wires:
  current_reference_generation/1(is_ref) -> [i_out_alphabeta_ref]  "i_out_inverter_pu_ref"
  dqpi_current_controller/1(u_out) -> u_ctrl_out/1, [u_ctrl_out]  "u_ctrl_out"
  [phase_grid] -> current_reference_generation/2(phase)
  inverter_current_output_pu_reference/1 -> current_reference_generation/1(mag_ref), [inverter_current_output_pu_reference]
  current_reference_generation/2(id_ref) -> dqpi_current_controller/1(id_ref)

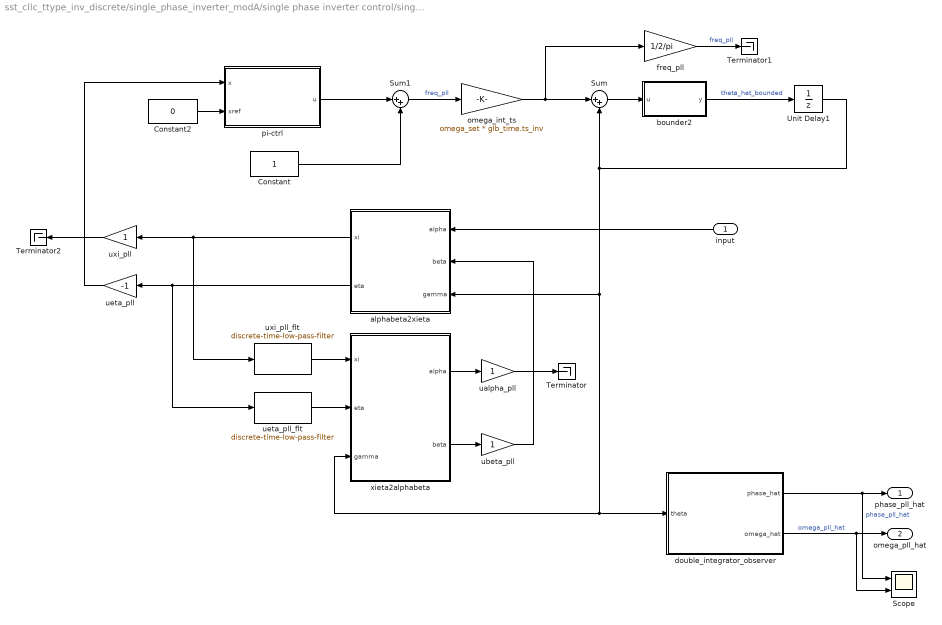
== system sst_cllc_ttype_inv_discrete/single_phase_inverter_modA/single phase inverter control/single_phase_inverter_ctrl/single_phase_pll ==
  input : Inport
  Constant : Constant
  Constant2 : Constant  Value=0
  Scope : Scope  NumInputPorts=2
      settings: ActiveDisplayYMinimum=-3.8846913322397336  ActiveDisplayYMaximum=3.9201093626393169
  Sum : Sum  Inputs=|++
  Sum1 : Sum  Inputs=|++
  Terminator : Terminator
  Terminator1 : Terminator
  Terminator2 : Terminator
  Unit Delay1 : UnitDelay  SampleTime=-1
  alphabeta2xieta : MATLAB Function  TreatAsAtomicUnit=on
  bounder2 : MATLAB Function  TreatAsAtomicUnit=on
  double_integrator_observer : Subsystem
  freq_pll : Gain  Gain=1/2/pi
  omega_int_ts : Gain  Gain=omega_set * glb_time.ts_inv
  pi-ctrl : Subsystem  mask{kp=1, ki=0, ts=glb_time.ts_inv, sat_pos=2, sat_neg=-2}
  ualpha_pll : Gain
  ubeta_pll : Gain
  ueta_pll : Gain  Gain=-1
  ueta_pll_flt : discrete_time_low_pass_filter/discrete-time-low-pass-filter  tau=2/omega_set  ts=glb_time.ts_inv
  uxi_pll : Gain
  uxi_pll_flt : discrete_time_low_pass_filter/discrete-time-low-pass-filter  tau=2/omega_set  ts=glb_time.ts_inv
  xieta2alphabeta : MATLAB Function  TreatAsAtomicUnit=on
  phase_pll_hat : Outport
  omega_pll_hat : Outport  Port=2
  wires:
  Sum/1 -> bounder2/1(u)
  alphabeta2xieta/1(xi) -> uxi_pll/1, uxi_pll_flt/1
  xieta2alphabeta/2(beta) -> ubeta_pll/1
  alphabeta2xieta/2(eta) -> ueta_pll/1, ueta_pll_flt/1
  omega_int_ts/1 -> freq_pll/1, Sum/1
  double_integrator_observer/1(phase_hat) -> Scope/1, phase_pll_hat/1  "phase_pll_hat"
  input/1 -> alphabeta2xieta/1(alpha)
  freq_pll/1 -> Terminator1/1  "freq_pll"
  ueta_pll_flt/1 -> xieta2alphabeta/2(eta)
  uxi_pll_flt/1 -> xieta2alphabeta/1(xi)
  ueta_pll/1 -> pi-ctrl/1(x)
  Sum1/1 -> omega_int_ts/1  "freq_pll"
  Constant2/1 -> pi-ctrl/2(xref)
  uxi_pll/1 -> Terminator2/1
  ubeta_pll/1 -> alphabeta2xieta/2(beta)
  xieta2alphabeta/1(alpha) -> ualpha_pll/1
  pi-ctrl/1(u) -> Sum1/1
  Constant/1 -> Sum1/2
  Unit Delay1/1 -> Sum/2, alphabeta2xieta/3(gamma), xieta2alphabeta/3(gamma), double_integrator_observer/1(theta)
  bounder2/1(y) -> Unit Delay1/1  "theta_hat_bounded"
  double_integrator_observer/2(omega_hat) -> Scope/2, omega_pll_hat/1  "omega_pll_hat"
  ualpha_pll/1 -> Terminator/1

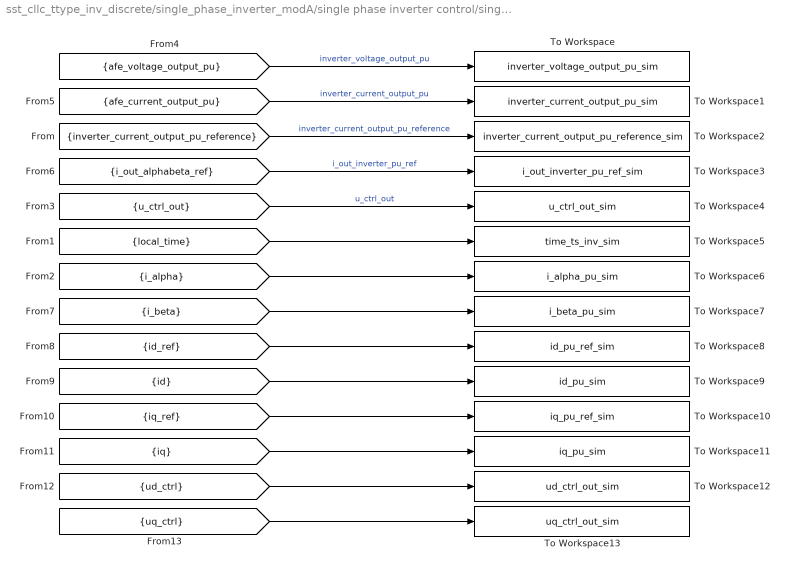
== system sst_cllc_ttype_inv_discrete/single_phase_inverter_modA/single phase inverter control/single_phase_inverter_ctrl/storage_data ==
  To Workspace : ToWorkspace  VariableName=inverter_voltage_output_pu_sim  SampleTime=-1
      settings: MaxDataPoints=glb_time.Ns_inv  Save2DSignal=2-D array (concatenate along first dimension)
  To Workspace1 : ToWorkspace  VariableName=inverter_current_output_pu_sim  SampleTime=-1
      settings: MaxDataPoints=glb_time.Ns_inv  Save2DSignal=2-D array (concatenate along first dimension)
  To Workspace10 : ToWorkspace  VariableName=iq_pu_ref_sim  SampleTime=-1
      settings: MaxDataPoints=glb_time.Ns_inv  Save2DSignal=2-D array (concatenate along first dimension)
  To Workspace11 : ToWorkspace  VariableName=iq_pu_sim  SampleTime=-1
      settings: MaxDataPoints=glb_time.Ns_inv  Save2DSignal=2-D array (concatenate along first dimension)
  To Workspace12 : ToWorkspace  VariableName=ud_ctrl_out_sim  SampleTime=-1
      settings: MaxDataPoints=glb_time.Ns_inv  Save2DSignal=2-D array (concatenate along first dimension)
  To Workspace13 : ToWorkspace  VariableName=uq_ctrl_out_sim  SampleTime=-1
      settings: MaxDataPoints=glb_time.Ns_inv  Save2DSignal=2-D array (concatenate along first dimension)
  To Workspace2 : ToWorkspace  VariableName=inverter_current_output_pu_reference_sim  SampleTime=-1
      settings: MaxDataPoints=glb_time.Ns_inv  Save2DSignal=2-D array (concatenate along first dimension)
  To Workspace3 : ToWorkspace  VariableName=i_out_inverter_pu_ref_sim  SampleTime=-1
      settings: MaxDataPoints=glb_time.Ns_inv  Save2DSignal=2-D array (concatenate along first dimension)
  To Workspace4 : ToWorkspace  VariableName=u_ctrl_out_sim  SampleTime=-1
      settings: MaxDataPoints=glb_time.Ns_inv  Save2DSignal=2-D array (concatenate along first dimension)
  To Workspace5 : ToWorkspace  VariableName=time_ts_inv_sim  SampleTime=-1
      settings: MaxDataPoints=glb_time.Ns_inv  Save2DSignal=2-D array (concatenate along first dimension)
  To Workspace6 : ToWorkspace  VariableName=i_alpha_pu_sim  SampleTime=-1
      settings: MaxDataPoints=glb_time.Ns_inv  Save2DSignal=2-D array (concatenate along first dimension)
  To Workspace7 : ToWorkspace  VariableName=i_beta_pu_sim  SampleTime=-1
      settings: MaxDataPoints=glb_time.Ns_inv  Save2DSignal=2-D array (concatenate along first dimension)
  To Workspace8 : ToWorkspace  VariableName=id_pu_ref_sim  SampleTime=-1
      settings: MaxDataPoints=glb_time.Ns_inv  Save2DSignal=2-D array (concatenate along first dimension)
  To Workspace9 : ToWorkspace  VariableName=id_pu_sim  SampleTime=-1
      settings: MaxDataPoints=glb_time.Ns_inv  Save2DSignal=2-D array (concatenate along first dimension)
  wires:
  [afe_voltage_output_pu] -> To Workspace/1  "inverter_voltage_output_pu"
  [afe_current_output_pu] -> To Workspace1/1  "inverter_current_output_pu"
  [inverter_current_output_pu_reference] -> To Workspace2/1  "inverter_current_output_pu_reference"
  [i_out_alphabeta_ref] -> To Workspace3/1  "i_out_inverter_pu_ref"
  [u_ctrl_out] -> To Workspace4/1  "u_ctrl_out"
  [local_time] -> To Workspace5/1
  [i_alpha] -> To Workspace6/1
  [i_beta] -> To Workspace7/1
  [id_ref] -> To Workspace8/1
  [id] -> To Workspace9/1
  [iq_ref] -> To Workspace10/1
  [iq] -> To Workspace11/1
  [ud_ctrl] -> To Workspace12/1
  [uq_ctrl] -> To Workspace13/1

== system sst_cllc_ttype_inv_discrete/single_phase_inverter_modB/single phase inverter control/single_phase_inverter_ctrl/scopes ==
  Bus Creator1 : BusCreator  Inputs=3
  Bus Creator2 : BusCreator  Inputs=2
  Bus Creator3 : BusCreator  Inputs=2
  Bus Creator4 : BusCreator  Inputs=2
  single phase inverter tracking current scope 1 : Scope  NumInputPorts=2
      settings: ActiveDisplayYMinimum=-1.23468017578125  ActiveDisplayYMaximum=1.23419189453125  DataLoggingVariableName=ScopeData12
  single phase inverter tracking current scope 2 : Scope  NumInputPorts=2
      settings: ActiveDisplayYMinimum=-1.2603759765625  ActiveDisplayYMaximum=1.2652587890625  DataLoggingVariableName=ScopeData2
  wires:
  Bus Creator4/1 -> single phase inverter tracking current scope 2/1  "i_load"
  [i_out_alphabeta_ref] -> Bus Creator4/1  "i_out_alphabeta_ref"
  [afe_current_output_pu] -> Bus Creator4/2  "inverter_current_output_pu"
  Bus Creator3/1 -> single phase inverter tracking current scope 2/2  "u_load"
  [afe_voltage_output_pu] -> Bus Creator3/2  "inverter_voltage_output_pu"
  [u_ctrl_out] -> Bus Creator3/1  "u_ctrl_out"
  [afe_current_output_pu] -> Bus Creator2/2  "inverter_current_output_pu"
  [inverter_current_output_pu_reference] -> Bus Creator1/1  "inverter_current_output_pu_reference"
  Bus Creator2/1 -> single phase inverter tracking current scope 1/1  "load"
  [afe_voltage_output_pu] -> Bus Creator2/1  "inverter_voltage_output_pu"
  [afe_current_output_pu] -> Bus Creator1/3  "inverter_current_output_pu"
  [i_out_alphabeta_ref] -> Bus Creator1/2  "i_out_inverter_pu_ref"
  Bus Creator1/1 -> single phase inverter tracking current scope 1/2  "is_tracking"

== system sst_cllc_ttype_inv_discrete/single_phase_inverter_modB/single phase inverter control/single_phase_inverter_ctrl/single_phase_current_control ==
  inverter_current_output_pu_reference : Inport
  current_reference_generation : Subsystem
  dqpi_current_controller : Subsystem
  u_ctrl_out : Outport
  tag scope: i_out_alphabeta_ref=scoped, inverter_current_output_pu_reference=scoped, u_ctrl_out=scoped
  wires:
  current_reference_generation/2(id_ref) -> dqpi_current_controller/1(id_ref)
  inverter_current_output_pu_reference/1 -> [inverter_current_output_pu_reference], current_reference_generation/1(mag_ref)
  [phase_grid] -> current_reference_generation/2(phase)
  dqpi_current_controller/1(u_out) -> [u_ctrl_out], u_ctrl_out/1  "u_ctrl_out"
  current_reference_generation/1(is_ref) -> [i_out_alphabeta_ref]  "i_out_inverter_pu_ref"

== system sst_cllc_ttype_inv_discrete/single_phase_inverter_modB/single phase inverter control/single_phase_inverter_ctrl/single_phase_pll ==
  input : Inport
  Constant : Constant
  Constant2 : Constant  Value=0
  Scope : Scope  NumInputPorts=2
      settings: ActiveDisplayYMinimum=-3.2854912154015015  ActiveDisplayYMaximum=3.4773424919151528
  Sum : Sum  Inputs=|++
  Sum1 : Sum  Inputs=|++
  Terminator : Terminator
  Terminator1 : Terminator
  Terminator2 : Terminator
  Unit Delay1 : UnitDelay  SampleTime=-1
  alphabeta2xieta : MATLAB Function  TreatAsAtomicUnit=on
  bounder2 : MATLAB Function  TreatAsAtomicUnit=on
  double_integrator_observer : Subsystem
  freq_pll : Gain  Gain=1/2/pi
  omega_int_ts : Gain  Gain=omega_set * glb_time.ts_inv
  pi-ctrl : Subsystem  mask{kp=1, ki=0, ts=glb_time.ts_inv, sat_pos=2, sat_neg=-2}
  ualpha_pll : Gain
  ubeta_pll : Gain
  ueta_pll : Gain  Gain=-1
  ueta_pll_flt : discrete_time_low_pass_filter/discrete-time-low-pass-filter  tau=2/omega_set  ts=glb_time.ts_inv
  uxi_pll : Gain
  uxi_pll_flt : discrete_time_low_pass_filter/discrete-time-low-pass-filter  tau=2/omega_set  ts=glb_time.ts_inv
  xieta2alphabeta : MATLAB Function  TreatAsAtomicUnit=on
  phase_pll_hat : Outport
  omega_pll_hat : Outport  Port=2
  wires:
  ualpha_pll/1 -> Terminator/1
  double_integrator_observer/2(omega_hat) -> omega_pll_hat/1, Scope/2  "omega_pll_hat"
  bounder2/1(y) -> Unit Delay1/1  "theta_hat_bounded"
  Unit Delay1/1 -> double_integrator_observer/1(theta), xieta2alphabeta/3(gamma), alphabeta2xieta/3(gamma), Sum/2
  Constant/1 -> Sum1/2
  pi-ctrl/1(u) -> Sum1/1
  xieta2alphabeta/1(alpha) -> ualpha_pll/1
  ubeta_pll/1 -> alphabeta2xieta/2(beta)
  uxi_pll/1 -> Terminator2/1
  Constant2/1 -> pi-ctrl/2(xref)
  Sum1/1 -> omega_int_ts/1  "freq_pll"
  ueta_pll/1 -> pi-ctrl/1(x)
  uxi_pll_flt/1 -> xieta2alphabeta/1(xi)
  ueta_pll_flt/1 -> xieta2alphabeta/2(eta)
  freq_pll/1 -> Terminator1/1  "freq_pll"
  input/1 -> alphabeta2xieta/1(alpha)
  double_integrator_observer/1(phase_hat) -> phase_pll_hat/1, Scope/1  "phase_pll_hat"
  omega_int_ts/1 -> Sum/1, freq_pll/1
  alphabeta2xieta/2(eta) -> ueta_pll_flt/1, ueta_pll/1
  xieta2alphabeta/2(beta) -> ubeta_pll/1
  alphabeta2xieta/1(xi) -> uxi_pll_flt/1, uxi_pll/1
  Sum/1 -> bounder2/1(u)

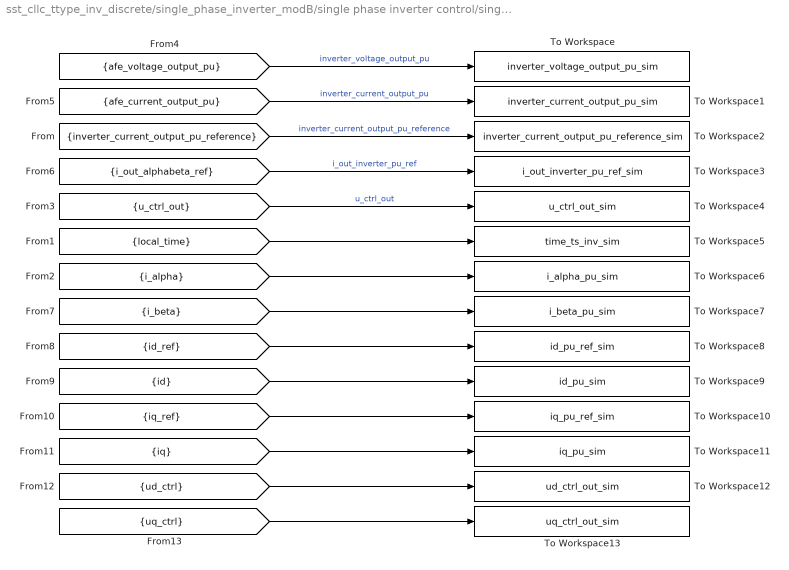
== system sst_cllc_ttype_inv_discrete/single_phase_inverter_modB/single phase inverter control/single_phase_inverter_ctrl/storage_data ==
  To Workspace : ToWorkspace  VariableName=inverter_voltage_output_pu_sim  SampleTime=-1
      settings: MaxDataPoints=glb_time.Ns_inv  Save2DSignal=2-D array (concatenate along first dimension)
  To Workspace1 : ToWorkspace  VariableName=inverter_current_output_pu_sim  SampleTime=-1
      settings: MaxDataPoints=glb_time.Ns_inv  Save2DSignal=2-D array (concatenate along first dimension)
  To Workspace10 : ToWorkspace  VariableName=iq_pu_ref_sim  SampleTime=-1
      settings: MaxDataPoints=glb_time.Ns_inv  Save2DSignal=2-D array (concatenate along first dimension)
  To Workspace11 : ToWorkspace  VariableName=iq_pu_sim  SampleTime=-1
      settings: MaxDataPoints=glb_time.Ns_inv  Save2DSignal=2-D array (concatenate along first dimension)
  To Workspace12 : ToWorkspace  VariableName=ud_ctrl_out_sim  SampleTime=-1
      settings: MaxDataPoints=glb_time.Ns_inv  Save2DSignal=2-D array (concatenate along first dimension)
  To Workspace13 : ToWorkspace  VariableName=uq_ctrl_out_sim  SampleTime=-1
      settings: MaxDataPoints=glb_time.Ns_inv  Save2DSignal=2-D array (concatenate along first dimension)
  To Workspace2 : ToWorkspace  VariableName=inverter_current_output_pu_reference_sim  SampleTime=-1
      settings: MaxDataPoints=glb_time.Ns_inv  Save2DSignal=2-D array (concatenate along first dimension)
  To Workspace3 : ToWorkspace  VariableName=i_out_inverter_pu_ref_sim  SampleTime=-1
      settings: MaxDataPoints=glb_time.Ns_inv  Save2DSignal=2-D array (concatenate along first dimension)
  To Workspace4 : ToWorkspace  VariableName=u_ctrl_out_sim  SampleTime=-1
      settings: MaxDataPoints=glb_time.Ns_inv  Save2DSignal=2-D array (concatenate along first dimension)
  To Workspace5 : ToWorkspace  VariableName=time_ts_inv_sim  SampleTime=-1
      settings: MaxDataPoints=glb_time.Ns_inv  Save2DSignal=2-D array (concatenate along first dimension)
  To Workspace6 : ToWorkspace  VariableName=i_alpha_pu_sim  SampleTime=-1
      settings: MaxDataPoints=glb_time.Ns_inv  Save2DSignal=2-D array (concatenate along first dimension)
  To Workspace7 : ToWorkspace  VariableName=i_beta_pu_sim  SampleTime=-1
      settings: MaxDataPoints=glb_time.Ns_inv  Save2DSignal=2-D array (concatenate along first dimension)
  To Workspace8 : ToWorkspace  VariableName=id_pu_ref_sim  SampleTime=-1
      settings: MaxDataPoints=glb_time.Ns_inv  Save2DSignal=2-D array (concatenate along first dimension)
  To Workspace9 : ToWorkspace  VariableName=id_pu_sim  SampleTime=-1
      settings: MaxDataPoints=glb_time.Ns_inv  Save2DSignal=2-D array (concatenate along first dimension)
  wires:
  [uq_ctrl] -> To Workspace13/1
  [ud_ctrl] -> To Workspace12/1
  [iq] -> To Workspace11/1
  [iq_ref] -> To Workspace10/1
  [id] -> To Workspace9/1
  [id_ref] -> To Workspace8/1
  [i_beta] -> To Workspace7/1
  [i_alpha] -> To Workspace6/1
  [local_time] -> To Workspace5/1
  [u_ctrl_out] -> To Workspace4/1  "u_ctrl_out"
  [i_out_alphabeta_ref] -> To Workspace3/1  "i_out_inverter_pu_ref"
  [inverter_current_output_pu_reference] -> To Workspace2/1  "inverter_current_output_pu_reference"
  [afe_current_output_pu] -> To Workspace1/1  "inverter_current_output_pu"
  [afe_voltage_output_pu] -> To Workspace/1  "inverter_voltage_output_pu"

== system sst_cllc_ttype_inv_discrete/single_phase_inverter_modA/single phase inverter control/single_phase_inverter_ctrl/single_phase_current_control/current_reference_generation ==
  mag_ref : Inport
  phase : Inport  Port=2
  Bus Creator : BusCreator  Inputs=2
  Product : Product
  Product1 : Product
  Sin : Trigonometry  Operator=cos
  Sin1 : Trigonometry
  is_ref : Outport
  id_ref : Outport  Port=2
  wires:
  Sin/1 -> Product/2
  phase/1 -> Sin1/1, Sin/1
  mag_ref/1 -> id_ref/1, Product1/1, Product/1
  Sin1/1 -> Product1/2
  Product/1 -> Bus Creator/1  "is_ref_alpha"
  Product1/1 -> Bus Creator/2  "is_ref_beta"
  Bus Creator/1 -> is_ref/1

== system sst_cllc_ttype_inv_discrete/single_phase_inverter_modA/single phase inverter control/single_phase_inverter_ctrl/single_phase_current_control/dqpi_current_controller ==
  id_ref : Inport
  Bus Creator : BusCreator  Inputs=3
  Bus Creator1 : BusCreator  Inputs=3
  alpha_beta currents : Scope  NumInputPorts=3
      settings: ActiveDisplayYMinimum=-0.89056396484375  ActiveDisplayYMaximum=0.93499755859375  DataLoggingVariableName=ScopeData2
  alphabeta2dq : Subsystem
  dq2alphabeta : Subsystem
  dq_vector_pi : Subsystem
  dq_vector_pi_tracking : Scope  NumInputPorts=2
      settings: ActiveDisplayYMinimum=-2.0541911300484528  ActiveDisplayYMaximum=1.5566373313135986  DataLoggingVariableName=ScopeData8
  i2alphabeta : Subsystem
  u_out : Outport
  tag scope: i_alpha=scoped, i_beta=scoped, id=scoped, id_ref=scoped, iq=scoped, ud_ctrl=scoped, uq_ctrl=scoped
  wires:
  dq2alphabeta/1(alpha) -> u_out/1
  id_ref/1 -> dq_vector_pi/1(id_ref), Bus Creator/1, [id_ref]
  alphabeta2dq/1("d ") -> Bus Creator/2, [id], dq_vector_pi/2(id)  "id"
  alphabeta2dq/2("q ") -> dq_vector_pi/3(iq), Bus Creator1/2, [iq]  "iq"
  [iq_ref] -> dq_vector_pi/4(iq_ref)
  Bus Creator1/1 -> dq_vector_pi_tracking/2
  Bus Creator/1 -> dq_vector_pi_tracking/1
  [ud_ctrl] -> Bus Creator/3
  [uq_ctrl] -> Bus Creator1/3
  [iq_ref] -> Bus Creator1/1
  [afe_current_output_pu] -> alpha_beta currents/1, i2alphabeta/1(i_alpha)  "i_load"
  i2alphabeta/1(i_alpha_out) -> alpha_beta currents/2, [i_alpha], alphabeta2dq/1(alpha)  "i_alpha"
  i2alphabeta/2(i_beta_out) -> [i_beta], alpha_beta currents/3, alphabeta2dq/2(beta)  "i_beta"
  dq_vector_pi/1(ud_ctrl) -> [ud_ctrl], dq2alphabeta/1(d)
  dq_vector_pi/2(uq_ctrl) -> [uq_ctrl], dq2alphabeta/2(q)

== system sst_cllc_ttype_inv_discrete/single_phase_inverter_modA/single phase inverter control/single_phase_inverter_ctrl/single_phase_pll/double_integrator_observer ==
  theta : Inport
  Gain : Gain  Gain=afe_ctrl.di_obs.Ldso  Multiplication=Matrix(K*u)
  Gain1 : Gain  Gain=afe_ctrl.di_obs.Adso  Multiplication=Matrix(K*u)
  Gain2 : Gain  Gain=afe_ctrl.di_obs.Cso  Multiplication=Matrix(K*u)
  Selector : Selector  InputPortWidth=2  IndexOptions=Index vector (dialog)  Indices=2  OutputSizes=1  RuntimeRangeChecks=off
  Sum : Sum  Inputs=-+|
  Sum1 : Sum  Inputs=|++
  Unit Delay : UnitDelay  SampleTime=-1
  bounder1 : MATLAB Function  TreatAsAtomicUnit=on
  bounder2 : MATLAB Function  TreatAsAtomicUnit=on
  kp3 : Gain  Gain=1/grid_emu.omega_grid_nom  SaturateOnIntegerOverflow=on  OutDataTypeStr=Inherit: Same as input  ParamDataTypeStr=Inherit: Same as input
  phase_hat : Outport
  omega_hat : Outport  Port=2
  wires:
  Gain/1 -> Sum1/1
  Gain2/1 -> bounder2/1(u)  "theta_hat"
  Gain1/1 -> Sum1/2
  Sum1/1 -> Unit Delay/1
  Sum/1 -> bounder1/1(u)  "e"
  Unit Delay/1 -> Selector/1, Gain1/1, Gain2/1
  theta/1 -> Sum/2  "theta"
  bounder1/1(y) -> Gain/1  "e_bounded"
  bounder2/1(y) -> phase_hat/1, Sum/1  "theta_hat_bounded"
  Selector/1 -> kp3/1
  kp3/1 -> omega_hat/1
